simulink model "YMBOX_Control_Core"  (R2024b)
settings: Solver=FixedStepDiscrete  StartTime=0.0  StopTime=3  RelTol=1e-3
PreLoadFcn:
  | run(fullfile(fileparts(get_param(bdroot,'FileName')), 'YMBOX_Deluxe_init.m'));
InitFcn:
  | YMBOX_InitializeModel('core',bdroot);
model workspace (MAT data in the model file):
  KuMDAS_ObserverBuildVariant : Simulink.Parameter (value not decoded)
undefined symbols (not defined in the file or in its folder): CeMDSM_DrvModeIfStart_enum, CeMDSM_DrvModeSpdSens_enum, CeMDSM_DrvModeSpdSmo_enum, CeMDSM_DrvModeTrq_enum, Cf_CONTROL_TASK_TIME_S, KbMDAS_SmoDeadTimeCompEnable_flg, KbMDSA_ActiveInverterCompEnable_flg, KbMDSA_UnifiedVoltageLimitEnable_flg, KbMDSP_DCBusVoltReportFilterEnable_flg, KbMDTM_DAxisPriorityInFW_flg, KbMDTM_FieldWeakeningEnable_flg, KbMDTM_FinalIqAntiWindupEnable_flg, KbMDTM_SensorlessFieldWeakeningEnable_flg, KbMDTM_TorquePriorityBelowBase_flg, KbMDTM_UnifiedConstraintEnable_flg, KfMDAS_ControlCountToElecRad_NULL, KfMDAS_IfAccel_rpms, KfMDAS_IfAlignTime_s, KfMDAS_IfBlendTime_s, KfMDAS_IfSwitchSpd_rpm, KfMDAS_NativeCountToMechRad_NULL, KfMDAS_ObserverExitRatio_NULL, KfMDAS_SlsCtrlPeriod_s, KfMDAS_SlsEAngleInit_rad, KfMDAS_SlsElecSpdMax_rads, KfMDAS_SlsElecSpdMin_rads, KfMDAS_SlsTwoPi_rad, KfMDAS_SmoAngleOffset_rad, KfMDAS_SmoCurrentZohCoefA_NULL, KfMDAS_SmoCurrentZohCoefB_AperV, KfMDAS_SmoDeadTimeCurrentBoundary_A, KfMDAS_SmoDeadTimeDuty_NULL, KfMDAS_SmoDeadTimePolarity_NULL, KfMDAS_SmoDeviceDrop_V, KfMDAS_SmoEmfLpfCoefA_NULL, KfMDAS_SmoEmfLpfCoefB_NULL, KfMDAS_SmoEmfLpfInvPole_s, KfMDAS_SmoErrBoundaryMax_A, KfMDAS_SmoErrBoundarySpan_A, KfMDAS_SmoGainSchedAlpha_NULL, KfMDAS_SmoGainSchedAngleComp_rad, KfMDAS_SmoGainSchedEmfLow_V, KfMDAS_SmoGainSchedInvSpan_PerV, KfMDAS_SmoLdMinusLq_H, KfMDAS_SmoPllKiTs_NULL, KfMDAS_SmoPllKp_NULL, KfMDAS_SmoPllMinEmf_V, KfMDAS_SmoPllSpeedLpfAlpha_NULL, KfMDAS_SmoSlideGainMin_V, KfMDAS_SmoSlideGainSpan_V, KfMDAS_SmoSwitchSpd_rpm, KfMDAS_SmoTotalDelay_s, KfMDCC_DqSoftwareOverCurrentThreshold_A, KfMDCC_PiKcTsId_NULL, KfMDCC_PiKcTsIq_NULL, KfMDCC_PiKiTsId_NULL, KfMDCC_PiKiTsIq_NULL, KfMDCC_PiKpValueId_NULL, KfMDCC_PiKpValueIq_NULL, KfMDCC_PwmFreq_Hz ... (+84)
libraries: YMBOX_SharedMath_Lib x11, spsabctoAlphaBetaZeroLib x1
(part 6 of 8)

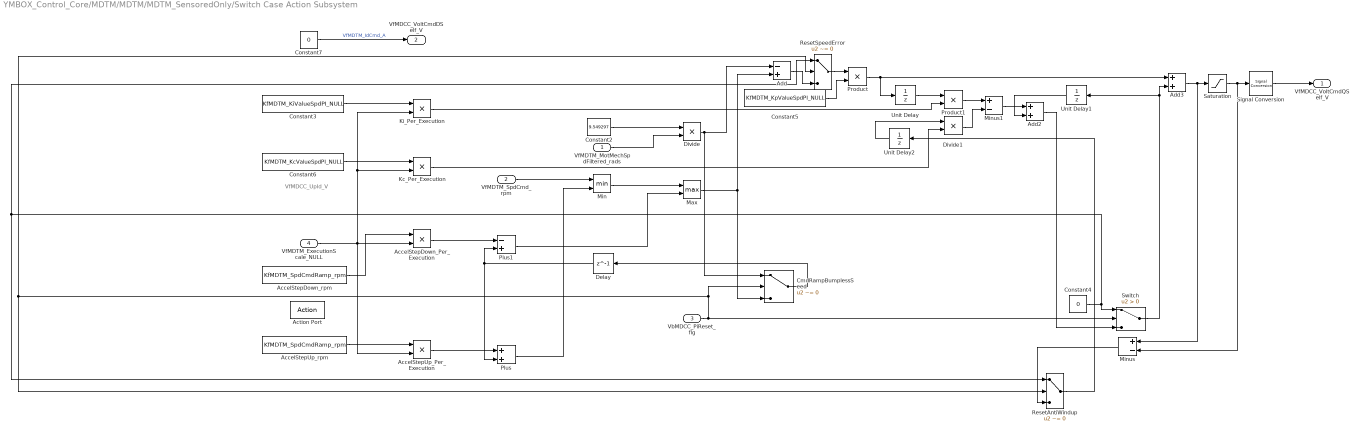
== system YMBOX_Control_Core/MDTM/MDTM/MDTM_SensoredOnly/Switch Case Action Subsystem ==
  note: VfMDCC_UpId_V
  VfMDTM_MotMechSpdFiltered_rads : Inport
  VfMDTM_SpdCmd_rpm : Inport  Port=2
  VbMDCC_PiReset_flg : Inport  Port=3
  VfMDTM_ExecutionScale_NULL : Inport  Port=4  OutDataTypeStr=single
  Action Port : ActionPort  InitializeStates=reset  ActionPortLabel=case [ 4 ]:
  AccelStepDown_Per_Execution : Product  Inputs=**
  AccelStepDown_rpm : Constant  Value=KfMDTM_SpdCmdRamp_rpm
  AccelStepUp_Per_Execution : Product  Inputs=**
  AccelStepUp_rpm : Constant  Value=KfMDTM_SpdCmdRamp_rpm
  Add : Sum  Inputs=-+
  Add2 : Sum  OutDataTypeStr=single
  Add3 : Sum
  CmdRampBumplessSeed : Switch  Criteria=u2 ~= 0  Threshold=0.5  SaturateOnIntegerOverflow=off  InputSameDT=off
  Constant2 : Constant  Value=9.549297  OutDataTypeStr=single
  Constant3 : Constant  Value=KfMDTM_KiValueSpdPI_NULL
  Constant4 : Constant  Value=0  OutDataTypeStr=single
  Constant5 : Constant  Value=KfMDTM_KpValueSpdPI_NULL
  Constant6 : Constant  Value=KfMDTM_KcValueSpdPI_NULL
  Constant7 : Constant  Value=0  OutDataTypeStr=single
  Delay : Delay  DelayLength=1
  Divide : Product  Inputs=**
  Divide1 : Product  Inputs=**
  Kc_Per_Execution : Product  Inputs=**
  Ki_Per_Execution : Product  Inputs=**
  Max : MinMax  Function=max  Inputs=2  OutDataTypeStr=single
  Min : MinMax  Inputs=2  OutDataTypeStr=single
  Minus : Sum  Inputs=+-
  Minus1 : Sum  Inputs=+-
  Plus : Sum
  Plus1 : Sum  Inputs=-+
  Product : Product
  Product1 : Product  RndMeth=Zero
  ResetAntiWindup : Switch  Criteria=u2 ~= 0
  ResetSpeedError : Switch  Criteria=u2 ~= 0
  Saturation : Saturate  UpperLimit=KfMDTM_IqCmdMax_A  LowerLimit=KfMDTM_IqCmdMin_A  OutDataTypeStr=single
  Signal Conversion : SignalConversion  OverrideOpt=off
  Switch : Switch  Criteria=u2 > Threshold  SaturateOnIntegerOverflow=off  InputSameDT=off
  Unit Delay : UnitDelay  SampleTime=-1  HasFrameUpgradeWarning=on
  Unit Delay1 : UnitDelay  SampleTime=-1  HasFrameUpgradeWarning=on
  Unit Delay2 : UnitDelay  SampleTime=-1  HasFrameUpgradeWarning=on
  VfMDCC_VoltCmdQSelf_V : Outport
  VfMDCC_VoltCmdDSelf_V : Outport  Port=2
  wires:
  Constant3/1 -> Ki_Per_Execution/1
  Kc_Per_Execution/1 -> Divide1/2
  Constant6/1 -> Kc_Per_Execution/1
  Constant7/1 -> VfMDCC_VoltCmdDSelf_V/1  "VfMDTM_IdCmd_A"
  VfMDTM_ExecutionScale_NULL/1 -> Ki_Per_Execution/2, Kc_Per_Execution/2, AccelStepDown_Per_Execution/2, AccelStepUp_Per_Execution/2
  AccelStepDown_rpm/1 -> AccelStepDown_Per_Execution/1
  Ki_Per_Execution/1 -> Product1/2
  AccelStepUp_rpm/1 -> AccelStepUp_Per_Execution/1
  AccelStepDown_Per_Execution/1 -> Plus1/1
  AccelStepUp_Per_Execution/1 -> Plus/1
  VfMDTM_SpdCmd_rpm/1 -> Min/1
  Plus1/1 -> Max/2
  Plus/1 -> Min/2
  Delay/1 -> Plus/2, Plus1/2
  Constant2/1 -> Divide/1
  VfMDTM_MotMechSpdFiltered_rads/1 -> Divide/2
  Min/1 -> Max/1
  Divide/1 -> CmdRampBumplessSeed/1, Add/1
  Max/1 -> CmdRampBumplessSeed/3, Add/2
  VbMDCC_PiReset_flg/1 -> ResetAntiWindup/2, ResetSpeedError/2, CmdRampBumplessSeed/2, Switch/2
  Add/1 -> ResetSpeedError/3
  Constant5/1 -> Product/2
  CmdRampBumplessSeed/1 -> Delay/1
  Product/1 -> Add3/1, Unit Delay/1
  Unit Delay2/1 -> Divide1/1
  Unit Delay/1 -> Product1/1
  Product1/1 -> Minus1/1
  Divide1/1 -> Minus1/2
  Minus1/1 -> Add2/1
  Add2/1 -> Switch/3
  Unit Delay1/1 -> Add2/2
  Constant4/1 -> ResetAntiWindup/1, ResetSpeedError/1, Switch/1
  Minus/1 -> ResetAntiWindup/3
  Switch/1 -> Add3/2, Unit Delay1/1
  Add3/1 -> Minus/1, Saturation/1
  Saturation/1 -> Signal Conversion/1, Minus/2
  Signal Conversion/1 -> VfMDCC_VoltCmdQSelf_V/1
  ResetSpeedError/1 -> Product/1
  ResetAntiWindup/1 -> Unit Delay2/1

== system YMBOX_Control_Core/MDTM/MDTM/MDTM_SensoredOnly/Switch Case Action Subsystem1 ==
  VfMDCC_TestUalphaUdId_NULL : Inport
  VfMDTM_TestUbetaUqIq_NULL : Inport  Port=2
  Action Port : ActionPort  ActionPortLabel=case [ 3 ]:
  Iq : Outport
  Id : Outport  Port=2
  wires:
  VfMDCC_TestUalphaUdId_NULL/1 -> Id/1
  VfMDTM_TestUbetaUqIq_NULL/1 -> Iq/1

== system YMBOX_Control_Core/MDTM/MDTM/MDTM_SensoredOnly/Switch Case Action Subsystem2 ==
  VfMDTM_TrqCmd_Nm : Inport
  Action Port : ActionPort  ActionPortLabel=case [ 5 ]:
  Constant7 : Constant  Value=0  OutDataTypeStr=single
  Gain : Gain  Gain=KfMDTM_Trq2Iq_NULL
  Iq : Outport
  Id : Outport  Port=2
  wires:
  Gain/1 -> Iq/1
  Constant7/1 -> Id/1  "VfMDTM_IdCmd_A"
  VfMDTM_TrqCmd_Nm/1 -> Gain/1

== system YMBOX_Control_Core/MDAS/MDAS_DriveModeRoute_Variant/MDAS_Route_SMO/Switch Case Action Subsystem/Switch Case Action Subsystem6 ==
  In1 : Inport
  Action Port : ActionPort  ActionPortLabel=if(u1 > KfPLL_HalfPositionCounts_NULL)
  Constant : Constant  Value=KfPLL_PositionCountsPerRev_NULL
  Minus : Sum  Inputs=+-
  Out1 : Outport
  wires:
  In1/1 -> Minus/1
  Constant/1 -> Minus/2
  Minus/1 -> Out1/1

== system YMBOX_Control_Core/MDAS/MDAS_DriveModeRoute_Variant/MDAS_Route_SMO/Switch Case Action Subsystem/Switch Case Action Subsystem7 ==
  In1 : Inport
  Action Port : ActionPort  ActionPortLabel=elseif(u1 < -KfPLL_HalfPositionCounts_NULL)
  Constant : Constant  Value=KfPLL_PositionCountsPerRev_NULL
  Minus : Sum
  Out1 : Outport
  wires:
  Minus/1 -> Out1/1
  In1/1 -> Minus/1
  Constant/1 -> Minus/2

== system YMBOX_Control_Core/MDAS/MDAS_DriveModeRoute_Variant/MDAS_Route_SMO/Switch Case Action Subsystem/Switch Case Action Subsystem8 ==
  In1 : Inport
  Action Port : ActionPort  ActionPortLabel=else
  Out1 : Outport
  wires:
  In1/1 -> Out1/1

== system YMBOX_Control_Core/MDAS/MDAS_DriveModeRoute_Variant/MDAS_Route_SensoredOnly/Sensored_AngleSpeed/Switch Case Action Subsystem6 ==
  In1 : Inport
  Action Port : ActionPort  ActionPortLabel=if(u1 > KfPLL_HalfPositionCounts_NULL)
  Constant : Constant  Value=KfPLL_PositionCountsPerRev_NULL
  Minus : Sum  Inputs=+-
  Out1 : Outport
  wires:
  Minus/1 -> Out1/1
  Constant/1 -> Minus/2
  In1/1 -> Minus/1

== system YMBOX_Control_Core/MDAS/MDAS_DriveModeRoute_Variant/MDAS_Route_SensoredOnly/Sensored_AngleSpeed/Switch Case Action Subsystem7 ==
  In1 : Inport
  Action Port : ActionPort  ActionPortLabel=elseif(u1 < -KfPLL_HalfPositionCounts_NULL)
  Constant : Constant  Value=KfPLL_PositionCountsPerRev_NULL
  Minus : Sum
  Out1 : Outport
  wires:
  Constant/1 -> Minus/2
  In1/1 -> Minus/1
  Minus/1 -> Out1/1

== system YMBOX_Control_Core/MDAS/MDAS_DriveModeRoute_Variant/MDAS_Route_SensoredOnly/Sensored_AngleSpeed/Switch Case Action Subsystem8 ==
  In1 : Inport
  Action Port : ActionPort  ActionPortLabel=else
  Out1 : Outport
  wires:
  In1/1 -> Out1/1

== system YMBOX_Control_Core/MDAS/Sensorless_FluxMRAS/Observer_Variant1_SMO/SMO_Observer/ExtendedEmfVoltageModel ==
  currentAb0_A : Inport
  appliedVoltageAb0_V : Inport  Port=2
  estimatedSpeed_rads : Inport  Port=3
  AlphaCrossCoupling : Product  Inputs=**
  BetaCrossCoupling : Product  Inputs=**
  CurrentAlphaBetaZero : Demux  Outputs=3
  EquivalentVoltageAb0 : Mux  Inputs=3
  ExtendedVoltageAlpha : Sum  Inputs=+-
  ExtendedVoltageBeta : Sum  Inputs=|++
  PreviousEstimatedSpeed : UnitDelay  InitialCondition=single(0)  SampleTime=-1
  PreviousMeasuredCurrent : UnitDelay  InitialCondition=single(0)  SampleTime=-1
  SpeedTimesLdMinusLq : Gain  Gain=KfMDAS_SmoLdMinusLq_H
  UnusedZeroSequenceCurrent : Terminator
  VoltageAlphaBetaZero : Demux  Outputs=3
  equivalentVoltageAb0_V : Outport
  wires:
  estimatedSpeed_rads/1 -> PreviousEstimatedSpeed/1
  appliedVoltageAb0_V/1 -> VoltageAlphaBetaZero/1
  CurrentAlphaBetaZero/2 -> AlphaCrossCoupling/2
  PreviousMeasuredCurrent/1 -> CurrentAlphaBetaZero/1
  currentAb0_A/1 -> PreviousMeasuredCurrent/1
  PreviousEstimatedSpeed/1 -> SpeedTimesLdMinusLq/1
  CurrentAlphaBetaZero/1 -> BetaCrossCoupling/2
  SpeedTimesLdMinusLq/1 -> BetaCrossCoupling/1, AlphaCrossCoupling/1
  CurrentAlphaBetaZero/3 -> UnusedZeroSequenceCurrent/1
  AlphaCrossCoupling/1 -> ExtendedVoltageAlpha/2
  BetaCrossCoupling/1 -> ExtendedVoltageBeta/2
  VoltageAlphaBetaZero/1 -> ExtendedVoltageAlpha/1
  VoltageAlphaBetaZero/2 -> ExtendedVoltageBeta/1
  VoltageAlphaBetaZero/3 -> EquivalentVoltageAb0/3
  ExtendedVoltageAlpha/1 -> EquivalentVoltageAb0/1
  ExtendedVoltageBeta/1 -> EquivalentVoltageAb0/2
  EquivalentVoltageAb0/1 -> equivalentVoltageAb0_V/1

== system YMBOX_Control_Core/MDAS/Sensorless_FluxMRAS/Observer_Variant1_SMO/SMO_Observer/PLL_Speed_Output ==
  IntegralSpeed_rads : Inport
  ProportionalCorrection_rads : Inport  Port=2
  CorrectedSpeed : Sum  OutDataTypeStr=single
  FilteredProportionalCorrection : Sum  OutDataTypeStr=single
  PreviousProportionalCorrection : UnitDelay  InitialCondition=single(0)  SampleTime=-1
  ProportionalFilterCoefficient : Gain  Gain=KfMDAS_SmoPllSpeedLpfAlpha_NULL  OutDataTypeStr=single
  ProportionalFilterError : Sum  Inputs=+-  OutDataTypeStr=single
  SpeedLimit : Saturate  UpperLimit=KfMDAS_SlsElecSpdMax_rads  LowerLimit=KfMDAS_SlsElecSpdMin_rads  OutDataTypeStr=single
  Speed_rads : Outport
  wires:
  CorrectedSpeed/1 -> SpeedLimit/1
  ProportionalCorrection_rads/1 -> ProportionalFilterError/1
  ProportionalFilterCoefficient/1 -> FilteredProportionalCorrection/1
  ProportionalFilterError/1 -> ProportionalFilterCoefficient/1
  PreviousProportionalCorrection/1 -> FilteredProportionalCorrection/2, ProportionalFilterError/2
  IntegralSpeed_rads/1 -> CorrectedSpeed/1
  FilteredProportionalCorrection/1 -> PreviousProportionalCorrection/1, CorrectedSpeed/2
  SpeedLimit/1 -> Speed_rads/1

== system YMBOX_Control_Core/MDAS/Sensorless_FluxMRAS/Observer_Variant1_SMO/SMO_Observer/SMO_SinCos_Adapter ==
  thetaRad : Inport
  twoPiRad : Inport  Port=2
  AnglePu_To_Single : DataTypeConversion  OutDataTypeStr=single
  Cos_To_ObserverType : DataTypeConversion  OutDataTypeStr=single
  SinCos_Service : YMBOX_SharedMath_Lib/SinCos_Service  SystemSampleTime=-1  VariantActivationTime=update diagram  AllowFlexibleInterface=on  Latency=0  AutoFrameSizeCalculation=off
  Sin_To_ObserverType : DataTypeConversion  OutDataTypeStr=single
  ThetaRad_To_Pu : Product  Inputs=*/
  cosTheta : Outport
  sinTheta : Outport  Port=2
  wires:
  Cos_To_ObserverType/1 -> cosTheta/1
  SinCos_Service/2 -> Sin_To_ObserverType/1
  thetaRad/1 -> ThetaRad_To_Pu/1
  twoPiRad/1 -> ThetaRad_To_Pu/2
  Sin_To_ObserverType/1 -> sinTheta/1
  SinCos_Service/1 -> Cos_To_ObserverType/1
  ThetaRad_To_Pu/1 -> AnglePu_To_Single/1
  AnglePu_To_Single/1 -> SinCos_Service/1

== system YMBOX_Control_Core/MDCC/MDCC_Subsystem/DqSoftwareOverCurrent_Diagnostic/CountWhenDqCurrentExceeded/AssertDqSoftwareOverCurrent ==
  Action Port : ActionPort  ActionPortLabel=else
  TRUE : Constant  OutDataTypeStr=boolean
  VbMDCC_DqSoftwareOverCurrent_flg : Outport  OutputWhenDisabled=reset  InitialOutput=false
  wires:
  TRUE/1 -> VbMDCC_DqSoftwareOverCurrent_flg/1

== system YMBOX_Control_Core/MDCC/MDCC_Subsystem/DqSoftwareOverCurrent_Diagnostic/CountWhenDqCurrentExceeded/IncrementDqSoftwareOverCurrentCount ==
  VuMDCC_DqSoftwareOverCurrentCount_cnt : Inport
  Action Port : ActionPort  ActionPortLabel=if(u1<u2)
  Constant : Constant  OutDataTypeStr=uint8
  Sum : Sum  OutDataTypeStr=uint8
  VuMDCC_DqSoftwareOverCurrentCountNew_cnt : Outport
  wires:
  VuMDCC_DqSoftwareOverCurrentCount_cnt/1 -> Sum/1
  Constant/1 -> Sum/2
  Sum/1 -> VuMDCC_DqSoftwareOverCurrentCountNew_cnt/1

== system YMBOX_Control_Core/MDCC/MDCC_Subsystem/DqSoftwareOverCurrent_Diagnostic/CountWhenDqCurrentNormal/DecrementDqSoftwareOverCurrentCount ==
  VuMDCC_DqSoftwareOverCurrentCount_cnt : Inport
  Action Port : ActionPort  ActionPortLabel=if(u1~=0)
  Constant : Constant  OutDataTypeStr=uint8
  Sum : Sum  Inputs=+-  OutDataTypeStr=uint8
  VuMDCC_DqSoftwareOverCurrentCountNew_cnt : Outport
  wires:
  Sum/1 -> VuMDCC_DqSoftwareOverCurrentCountNew_cnt/1
  Constant/1 -> Sum/2
  VuMDCC_DqSoftwareOverCurrentCount_cnt/1 -> Sum/1

== system YMBOX_Control_Core/MDCC/MDCC_Subsystem/UdUqCalc/UdUqCalc/PI_Id_Self ==
  note: VfMDCC_UpId_V
  VfMDCC_DCurCmd_A : Inport
  VfMDCC_DCur_A : Inport  Port=2
  VfMDCC_PiKpValueId_NULL : Inport  Port=3
  VbMDCC_PiReset_flg : Inport  Port=4
  VfMDCC_k_effective_NULL : Inport  Port=5
  Add : Sum  Inputs=+-
  Add1 : Sum
  Add2 : Sum  OutDataTypeStr=single
  Add3 : Sum
  Constant : Constant  Value=KfMDCC_PiKiTsId_NULL
  Constant1 : Constant  Value=KfMDCC_PiKcTsId_NULL
  Constant2 : Constant  Value=0  OutDataTypeStr=single
  Constant3 : Constant  OutDataTypeStr=single
  Delay : Delay  DelayLength=1  InputProcessing=Columns as channels (frame based)
  Divide2 : Product  Inputs=**
  Plus : Sum  Inputs=-+
  Product : Product
  Product1 : Product  RndMeth=Zero
  Product2 : Product  OutDataTypeStr=single  RndMeth=Zero
  Switch : Switch  Criteria=u2 > Threshold  SaturateOnIntegerOverflow=off  InputSameDT=off
  Unit Delay : UnitDelay  SampleTime=-1  HasFrameUpgradeWarning=on
  Unit Delay1 : UnitDelay  SampleTime=-1  HasFrameUpgradeWarning=on
  VfMDCC_VoltCmdDSelf_V : Outport
  wires:
  Divide2/1 -> Product2/1
  Plus/1 -> Divide2/2
  Constant3/1 -> Plus/1
  VfMDCC_k_effective_NULL/1 -> Plus/2
  Delay/1 -> Divide2/1
  Add2/1 -> Switch/3
  VbMDCC_PiReset_flg/1 -> [VbMDCC_PiReset_flg]
  Switch/1 -> Unit Delay1/1, Add3/2
  Constant2/1 -> Switch/1
  [VbMDCC_PiReset_flg] -> Switch/2
  Constant1/1 -> Product2/2
  Add3/1 -> VfMDCC_VoltCmdDSelf_V/1, Delay/1
  Unit Delay1/1 -> Add2/2
  Add1/1 -> Add2/1
  Constant/1 -> Product1/2
  Unit Delay/1 -> Product1/1
  Product/1 -> Add3/1, Unit Delay/1
  VfMDCC_PiKpValueId_NULL/1 -> Product/2
  Add/1 -> Product/1
  VfMDCC_DCur_A/1 -> Add/2
  VfMDCC_DCurCmd_A/1 -> Add/1
  Product1/1 -> Add1/1
  Product2/1 -> Add1/2

== system YMBOX_Control_Core/MDCC/MDCC_Subsystem/UdUqCalc/UdUqCalc/PI_Iq_Self ==
  note: VfMDCC_UpIq_V
  VfMDCC_QCurCmd_A : Inport
  VfMDCC_QCur_A : Inport  Port=2
  VfMDCC_PiKpValueIq_NULL : Inport  Port=3
  VbMDCC_PiReset_flg : Inport  Port=4
  VfMDCC_k_effective_NULL : Inport  Port=5
  Add : Sum  Inputs=+-
  Add1 : Sum  OutDataTypeStr=single
  Add2 : Sum  OutDataTypeStr=single
  Add3 : Sum
  Constant : Constant  Value=KfMDCC_PiKiTsIq_NULL
  Constant1 : Constant  Value=KfMDCC_PiKcTsIq_NULL
  Constant2 : Constant  Value=0  OutDataTypeStr=single
  Constant3 : Constant  OutDataTypeStr=single
  Delay : Delay  DelayLength=1  InputProcessing=Columns as channels (frame based)
  Divide2 : Product  Inputs=**
  Plus : Sum  Inputs=-+
  Product : Product
  Product1 : Product  RndMeth=Zero
  Product2 : Product  OutDataTypeStr=single  RndMeth=Zero
  Switch : Switch  Criteria=u2 > Threshold  SaturateOnIntegerOverflow=off  InputSameDT=off
  Unit Delay : UnitDelay  SampleTime=-1  HasFrameUpgradeWarning=on
  Unit Delay1 : UnitDelay  SampleTime=-1  HasFrameUpgradeWarning=on
  VfMDCC_VoltCmdQSelf_V : Outport
  wires:
  Plus/1 -> Divide2/2
  Divide2/1 -> Product2/1
  VfMDCC_k_effective_NULL/1 -> Plus/2
  Constant3/1 -> Plus/1
  Delay/1 -> Divide2/1
  Switch/1 -> Unit Delay1/1, Add3/2
  Add2/1 -> Switch/3
  Constant2/1 -> Switch/1
  [VbMDCC_PiReset_flg] -> Switch/2
  VbMDCC_PiReset_flg/1 -> [VbMDCC_PiReset_flg]
  Constant1/1 -> Product2/2
  Add3/1 -> Delay/1, VfMDCC_VoltCmdQSelf_V/1
  Unit Delay1/1 -> Add2/2
  Add1/1 -> Add2/1
  Constant/1 -> Product1/2
  Unit Delay/1 -> Product1/1
  Product/1 -> Add3/1, Unit Delay/1
  VfMDCC_PiKpValueIq_NULL/1 -> Product/2
  Add/1 -> Product/1
  VfMDCC_QCur_A/1 -> Add/2
  VfMDCC_QCurCmd_A/1 -> Add/1
  Product1/1 -> Add1/1
  Product2/1 -> Add1/2

== system YMBOX_Control_Core/MDCC/MDCC_Subsystem/UdUqCalc/UdUqCalc/Switch Case Action Subsystem ==
  VfMDCC_VoltCmdDSelf_V : Inport
  VfMDCC_VoltCmdQSelf_V : Inport  Port=2
  Action Port : ActionPort  ActionPortLabel=case [ 0 ]:
  VfMDCC_VoltD_V : Outport
  VfMDCC_VoltQ_V : Outport  Port=2
  wires:
  VfMDCC_VoltCmdDSelf_V/1 -> VfMDCC_VoltD_V/1
  VfMDCC_VoltCmdQSelf_V/1 -> VfMDCC_VoltQ_V/1

== system YMBOX_Control_Core/MDCC/MDCC_Subsystem/UdUqCalc/UdUqCalc/Switch Case Action Subsystem1 ==
  VfMDCC_VoltCmdDSelf_V : Inport
  VfMDCC_VoltCmdQSelf_V : Inport  Port=2
  VfMDCC_DCur_A : Inport  Port=3
  VfMDCC_QCur_A : Inport  Port=4
  VfMDCC_MotESpdFiltered_rads : Inport  Port=5
  Action Port : ActionPort  ActionPortLabel=case [ 1 ]:
  Add : Sum
  Add1 : Sum
  Add2 : Sum  Inputs=+-
  Constant : Constant  Value=KfMDMP_EquiInductanceValueD_H
  Constant1 : Constant  Value=KfMDMP_EquiFluxValue_Wb
  Constant2 : Constant  Value=KfMDCC_VqFFScale_NULL
  Constant3 : Constant  Value=KfMDMP_EquiInductanceValueQ_H
  Constant4 : Constant  Value=KfMDCC_VdFFScale_NULL
  Product{,1..2,5} (4 alike) : Product
  Product3 : Product  RndMeth=Zero
  Product4 : Product  RndMeth=Zero
  VfMDCC_VoltD_V : Outport
  VfMDCC_VoltQ_V : Outport  Port=2
  wires:
  Constant/1 -> Product/1
  Constant1/1 -> Add/2
  Constant3/1 -> Product3/2
  Product4/1 -> Product5/1
  Add1/1 -> VfMDCC_VoltQ_V/1
  Product1/1 -> Product2/1
  Constant4/1 -> Product5/2
  Constant2/1 -> Product2/2
  VfMDCC_VoltCmdQSelf_V/1 -> Add1/1
  Product5/1 -> Add2/2
  VfMDCC_DCur_A/1 -> Product/2
  Product/1 -> Add/1
  VfMDCC_QCur_A/1 -> Product3/1
  Add/1 -> Product1/2
  Add2/1 -> VfMDCC_VoltD_V/1
  VfMDCC_MotESpdFiltered_rads/1 -> Product4/2, Product1/1
  Product3/1 -> Product4/1
  Product2/1 -> Add1/2
  VfMDCC_VoltCmdDSelf_V/1 -> Add2/1

== system YMBOX_Control_Core/MDCC/MDCC_Subsystem/UdUqCalc/UdUqCalc/Switch Case Action Subsystem2 ==
  VfMDCC_VoltCmdDSelf_V : Inport
  VfMDCC_VoltCmdQSelf_V : Inport  Port=2
  VfMDCC_QCur_A : Inport  Port=3
  VfMDCC_MotESpdFiltered_rads : Inport  Port=4
  Action Port : ActionPort  ActionPortLabel=case [ 2 ]:
  Add2 : Sum  Inputs=+-
  Constant3 : Constant  Value=KfMDMP_EquiInductanceValueQ_H
  Constant4 : Constant  Value=KfMDCC_VdFFScale_NULL
  Product3 : Product  RndMeth=Zero
  Product4 : Product  RndMeth=Zero
  Product5 : Product
  VfMDCC_VoltD_V : Outport
  VfMDCC_VoltQ_V : Outport  Port=2
  wires:
  Product4/1 -> Product5/1
  VfMDCC_VoltCmdDSelf_V/1 -> Add2/1
  VfMDCC_VoltCmdQSelf_V/1 -> VfMDCC_VoltQ_V/1
  Constant3/1 -> Product3/2
  Product5/1 -> Add2/2
  Product3/1 -> Product4/1
  VfMDCC_MotESpdFiltered_rads/1 -> Product4/2
  Add2/1 -> VfMDCC_VoltD_V/1
  VfMDCC_QCur_A/1 -> Product3/1
  Constant4/1 -> Product5/2

== system YMBOX_Control_Core/MDCC/MDCC_Subsystem/UdUqCalc/UdUqCalc/Switch Case Action Subsystem3 ==
  VfMDCC_VoltCmdDSelf_V : Inport
  VfMDCC_VoltCmdQSelf_V : Inport  Port=2
  VfMDCC_DCur_A : Inport  Port=3
  VfMDCC_MotESpdFiltered_rads : Inport  Port=4
  Action Port : ActionPort  ActionPortLabel=case [ 3 ]:
  Add : Sum
  Add1 : Sum
  Constant : Constant  Value=KfMDMP_EquiInductanceValueD_H
  Constant1 : Constant  Value=KfMDMP_EquiFluxValue_Wb
  Constant2 : Constant  Value=KfMDCC_VqFFScale_NULL
  Product : Product
  Product1 : Product
  Product2 : Product
  VfMDCC_VoltD_V : Outport
  VfMDCC_VoltQ_V : Outport  Port=2
  wires:
  VfMDCC_MotESpdFiltered_rads/1 -> Product1/1
  VfMDCC_DCur_A/1 -> Product/2
  Product/1 -> Add/1
  Add1/1 -> VfMDCC_VoltQ_V/1
  Product1/1 -> Product2/1
  VfMDCC_VoltCmdQSelf_V/1 -> Add1/1
  Constant1/1 -> Add/2
  Constant/1 -> Product/1
  Product2/1 -> Add1/2
  VfMDCC_VoltCmdDSelf_V/1 -> VfMDCC_VoltD_V/1
  Add/1 -> Product1/2
  Constant2/1 -> Product2/2

== system YMBOX_Control_Core/MDSA/MDSA_Subsystem/PwmOutput/PwmEnable/SVM ==
  VfMDSA_VoltAlpha_V : Inport
  VfMDSA_VoltBeta_V : Inport  Port=2
  VfMDSA_DCBusVolt_V : Inport  Port=3
  SectorCalc : Subsystem  RTWFcnName=vPwm_MDSA_SVM_SectorCalc  RTWFileName=MDSA
      settings: RTWSystemCode=Nonreusable function  RTWFcnNameOpts=User specified  RTWFileNameOpts=User specified
  T1T2CoefCalc : Subsystem  RTWFcnName=vPwm_MDSA_SVM_T1T2CoefCalc  RTWFileName=MDSA
      settings: RTWSystemCode=Nonreusable function  RTWFcnNameOpts=User specified  RTWFileNameOpts=User specified
  TonUVWCal : Subsystem  RTWFcnName=vPwm_MDSA_SVM_TonUVWCalc  RTWFileName=MDSA
      settings: RTWSystemCode=Nonreusable function  RTWFcnNameOpts=User specified  RTWFileNameOpts=User specified
  VfMDSA_PwmDutyCyclePhaseU_NULL : Outport
  VfMDSA_PwmDutyCyclePhaseV_NULL : Outport  Port=2
  VfMDSA_PwmDutyCyclePhaseW_NULL : Outport  Port=3
  VfMDSA_k_svm_NULL : Outport  Port=4
  wires:
  T1T2CoefCalc/3(VfMDSA_k_svm_NULL) -> VfMDSA_k_svm_NULL/1
  TonUVWCal/1(VfMDSA_PwmDutyCyclePhaseU_NULL) -> VfMDSA_PwmDutyCyclePhaseU_NULL/1
  TonUVWCal/3(VfMDSA_PwmDutyCyclePhaseW_NULL) -> VfMDSA_PwmDutyCyclePhaseW_NULL/1
  TonUVWCal/2(VfMDSA_PwmDutyCyclePhaseV_NULL) -> VfMDSA_PwmDutyCyclePhaseV_NULL/1
  SectorCalc/1(VeMDSA_Sector_enum) -> TonUVWCal/1(VeMDSA_Sector_enum), T1T2CoefCalc/1(VeMDSA_Sector_enum)
  T1T2CoefCalc/2(VfMDSA_T2Coef_NULL) -> TonUVWCal/3(VfMDSA_T2Coef_NULL)
  T1T2CoefCalc/1(VfMDSA_T1Coef_NULL) -> TonUVWCal/2(VfMDSA_T1Coef_NULL)
  VfMDSA_DCBusVolt_V/1 -> T1T2CoefCalc/4(VfMDSA_DCBusVolt_V)
  VfMDSA_VoltBeta_V/1 -> SectorCalc/2(VfMDSA_VoltBeta_V), T1T2CoefCalc/3(VfMDSA_VoltBeta_V)
  VfMDSA_VoltAlpha_V/1 -> SectorCalc/1(VfMDSA_VoltAlpha_V), T1T2CoefCalc/2(VfMDSA_VoltAlpha_V)

== system YMBOX_Control_Core/MDSA/MDSA_Subsystem/UalphaUbetaCalc/Subsystem/UalphaUbetaCalc1 ==
  VfMDSA_VoltD_V : Inport
  VfMDSA_VoltQ_V : Inport  Port=2
  VfMDSA_MotElecAngle_rad : Inport  Port=3
  VfMDSA_MotElecSpd_rads : Inport  Port=4
  VfMDSA_PwmFreq_Hz : Inport  Port=5
  Action Port : ActionPort  ActionPortLabel=default:
  ElecAngle_Advance_SinCos : Subsystem  TreatAsAtomicUnit=on  RTWFcnName=vPwm_MDSA_UalphaUbetaCalc1_LookUpEAngleEstimatedCosSin  RTWFileName=MDSA
      settings: RTWFcnNameOpts=User specified  RTWFileNameOpts=User specified
  IPark : Subsystem  TreatAsAtomicUnit=on  RTWFcnName=vPwm_MDSA_UalphaUbetaCalc1_IPark  RTWFileName=MDSA
      settings: RTWFcnNameOpts=User specified  RTWFileNameOpts=User specified
  VfMDSA_VoltAlpha_V : Outport
  VfMDSA_VoltBeta_V : Outport  Port=2
  wires:
  VfMDSA_PwmFreq_Hz/1 -> ElecAngle_Advance_SinCos/3(VfMDSA_PwmFreq_Hz)
  IPark/2(VfMDSA_VoltBeta_V) -> VfMDSA_VoltBeta_V/1
  IPark/1(VfMDSA_VoltAlpha_V) -> VfMDSA_VoltAlpha_V/1
  VfMDSA_VoltD_V/1 -> IPark/1(VfMDSA_VoltD_V)  "VfMDSA_VoltD_V"
  VfMDSA_VoltQ_V/1 -> IPark/2(VfMDSA_VoltQ_V)  "VfMDSA_VoltQ_V"
  ElecAngle_Advance_SinCos/2(VfMDSA_EAngleEstimatedSin_NULL) -> IPark/4(VfMDSA_EAngleEstimatedSin_NULL)
  ElecAngle_Advance_SinCos/1(VfMDSA_EAngleEstimatedCos_NULL) -> IPark/3(VfMDSA_EAngleEstimatedCos_NULL)
  VfMDSA_MotElecSpd_rads/1 -> ElecAngle_Advance_SinCos/2(VfMDSA_MotElecSpd_rads)
  VfMDSA_MotElecAngle_rad/1 -> ElecAngle_Advance_SinCos/1(VfMDSA_MotElecAngle_rad)

== system YMBOX_Control_Core/MDSA/MDSA_Subsystem/UalphaUbetaCalc/Subsystem/UalphaUbetaCalc2 ==
  VfMDSA_TestUalphaUdId_NULL : Inport
  VfMDSA_TestUbetaUqIq_NULL : Inport  Port=2
  Action Port : ActionPort  ActionPortLabel=case [ 1 ]:
  VfMDSA_VoltAlpha_V : Outport
  VfMDSA_VoltBeta_V : Outport  Port=2
  wires:
  VfMDSA_TestUbetaUqIq_NULL/1 -> VfMDSA_VoltBeta_V/1
  VfMDSA_TestUalphaUdId_NULL/1 -> VfMDSA_VoltAlpha_V/1

== system YMBOX_Control_Core/MDTM/MDTM/MDTM_SMO/SMO_Handover_Current_Comp/Current_Vector_Crossfade ==
  sourceId : Inport  OutDataTypeStr=single
  sourceIq : Inport  Port=2  OutDataTypeStr=single
  currentWeight : Inport  Port=3  OutDataTypeStr=single
  targetId : Inport  Port=4  OutDataTypeStr=single
  targetIq : Inport  Port=5  OutDataTypeStr=single
  Active_Blend_Enable : EnablePort  OutDataTypeStr=boolean
  Blend_Id : Sum  Inputs=|++
  Blend_Iq : Sum  Inputs=|++
  One_Minus_Current_Weight : Sum  Inputs=+-
  Unity : Constant  Value=single(1)
  Weighted_Source_Id : Product  Inputs=**
  Weighted_Source_Iq : Product  Inputs=**
  Weighted_Target_Id : Product  Inputs=**
  Weighted_Target_Iq : Product  Inputs=**
  idBlend : Outport  OutDataTypeStr=single
  iqBlend : Outport  Port=2  OutDataTypeStr=single
  wires:
  Blend_Iq/1 -> iqBlend/1
  Blend_Id/1 -> idBlend/1
  Weighted_Target_Iq/1 -> Blend_Iq/2
  Weighted_Source_Iq/1 -> Blend_Iq/1
  targetIq/1 -> Weighted_Target_Iq/1
  sourceIq/1 -> Weighted_Source_Iq/1
  Weighted_Target_Id/1 -> Blend_Id/2
  Weighted_Source_Id/1 -> Blend_Id/1
  targetId/1 -> Weighted_Target_Id/1
  One_Minus_Current_Weight/1 -> Weighted_Source_Id/2, Weighted_Source_Iq/2
  sourceId/1 -> Weighted_Source_Id/1
  currentWeight/1 -> One_Minus_Current_Weight/2, Weighted_Target_Id/2, Weighted_Target_Iq/2
  Unity/1 -> One_Minus_Current_Weight/1

== system YMBOX_Control_Core/MDTM/MDTM/MDTM_SMO/SMO_Handover_Current_Comp/Handover_Enable_Logic ==
  modeCmd : Inport  OutDataTypeStr=uint16
  modeReq : Inport  Port=2  OutDataTypeStr=uint16
  blendWeight : Inport  Port=3  OutDataTypeStr=single
  Blend_Complete : Constant  Value=single(1)
  Enable_Active_Blend : Logic  Inputs=3  IconShape=distinctive
  Is_Blend_Incomplete : RelationalOperator  Operator=<
  Is_Mode_17 : RelationalOperator  Operator===
  Is_Request_6 : RelationalOperator  Operator===
  Mode_SMO_ClosedLoop : Constant  Value=uint16(17)
  Request_Product_SMO : Constant  Value=uint16(6)
  activeBlend : Outport  OutDataTypeStr=boolean
  wires:
  Enable_Active_Blend/1 -> activeBlend/1
  Is_Blend_Incomplete/1 -> Enable_Active_Blend/3
  Is_Request_6/1 -> Enable_Active_Blend/2
  Is_Mode_17/1 -> Enable_Active_Blend/1
  Blend_Complete/1 -> Is_Blend_Incomplete/2
  blendWeight/1 -> Is_Blend_Incomplete/1
  Request_Product_SMO/1 -> Is_Request_6/2
  modeReq/1 -> Is_Request_6/1
  Mode_SMO_ClosedLoop/1 -> Is_Mode_17/2
  modeCmd/1 -> Is_Mode_17/1

== system YMBOX_Control_Core/MDTM/MDTM/MDTM_SMO/SMO_Handover_Current_Comp/Source_Frame_Rotation ==
  sourceId0 : Inport  OutDataTypeStr=single
  sourceIq0 : Inport  Port=2  OutDataTypeStr=single
  blendWeight : Inport  Port=3  OutDataTypeStr=single
  elecAngleDeltaRad : Inport  Port=4  OutDataTypeStr=single
  Active_Blend_Enable : EnablePort  OutDataTypeStr=boolean
  Id_Cos : Product  Inputs=**
  Id_Sin : Product  Inputs=**
  Iq_Cos : Product  Inputs=**
  Iq_Sin : Product  Inputs=**
  Rotated_Source_Id : Sum  Inputs=+-
  Rotated_Source_Iq : Sum  Inputs=|++
  SourcePhase_PU_Floor : Rounding
  SourcePhase_PU_Wrap : Sum  Inputs=+-
  SourcePhase_RadToPU : Gain  Gain=single(0.15915494)
  SourcePhase_SinCos_Service : YMBOX_SharedMath_Lib/SinCos_Service  SystemSampleTime=-1  VariantActivationTime=update diagram  AllowFlexibleInterface=on  Latency=0  AutoFrameSizeCalculation=off
  Source_Phase : Product  Inputs=**
  sourceId : Outport  OutDataTypeStr=single
  sourceIq : Outport  Port=2  OutDataTypeStr=single
  wires:
  blendWeight/1 -> Source_Phase/1
  SourcePhase_PU_Wrap/1 -> SourcePhase_SinCos_Service/1
  elecAngleDeltaRad/1 -> Source_Phase/2
  SourcePhase_RadToPU/1 -> SourcePhase_PU_Wrap/1, SourcePhase_PU_Floor/1
  Source_Phase/1 -> SourcePhase_RadToPU/1
  sourceIq0/1 -> Iq_Sin/1, Iq_Cos/1
  sourceId0/1 -> Id_Cos/1, Id_Sin/1
  SourcePhase_SinCos_Service/1 -> Iq_Cos/2, Id_Cos/2
  SourcePhase_SinCos_Service/2 -> Id_Sin/2, Iq_Sin/2
  Id_Sin/1 -> Rotated_Source_Iq/1
  Iq_Cos/1 -> Rotated_Source_Iq/2
  Id_Cos/1 -> Rotated_Source_Id/1
  Iq_Sin/1 -> Rotated_Source_Id/2
  Rotated_Source_Iq/1 -> sourceIq/1
  Rotated_Source_Id/1 -> sourceId/1
  SourcePhase_PU_Floor/1 -> SourcePhase_PU_Wrap/2

== system YMBOX_Control_Core/MDTM/MDTM/MDTM_SMO/SMO_Handover_Current_Comp/Target_Frame_Rotation ==
  idRaw : Inport  OutDataTypeStr=single
  iqRaw : Inport  Port=2  OutDataTypeStr=single
  blendWeight : Inport  Port=3  OutDataTypeStr=single
  elecAngleDeltaRad : Inport  Port=4  OutDataTypeStr=single
  Active_Blend_Enable : EnablePort  OutDataTypeStr=boolean
  Id_Cos : Product  Inputs=**
  Id_Sin : Product  Inputs=**
  Iq_Cos : Product  Inputs=**
  Iq_Sin : Product  Inputs=**
  One_Minus_Blend : Sum  Inputs=+-
  Rotated_Target_Id : Sum  Inputs=+-
  Rotated_Target_Iq : Sum  Inputs=|++
  TargetPhase_PU_Floor : Rounding
  TargetPhase_PU_Wrap : Sum  Inputs=+-
  TargetPhase_RadToPU : Gain  Gain=single(0.15915494)
  TargetPhase_SinCos_Service : YMBOX_SharedMath_Lib/SinCos_Service  SystemSampleTime=-1  VariantActivationTime=update diagram  AllowFlexibleInterface=on  Latency=0  AutoFrameSizeCalculation=off
  Target_Phase_Magnitude : Product  Inputs=**
  Target_Phase_Negate : Gain  Gain=single(-1)
  Unity : Constant  Value=single(1)
  targetId : Outport  OutDataTypeStr=single
  targetIq : Outport  Port=2  OutDataTypeStr=single
  wires:
  One_Minus_Blend/1 -> Target_Phase_Magnitude/1
  Unity/1 -> One_Minus_Blend/1
  Target_Phase_Magnitude/1 -> Target_Phase_Negate/1
  blendWeight/1 -> One_Minus_Blend/2
  elecAngleDeltaRad/1 -> Target_Phase_Magnitude/2
  Target_Phase_Negate/1 -> TargetPhase_RadToPU/1
  TargetPhase_RadToPU/1 -> TargetPhase_PU_Wrap/1, TargetPhase_PU_Floor/1
  TargetPhase_PU_Wrap/1 -> TargetPhase_SinCos_Service/1
  idRaw/1 -> Id_Cos/1, Id_Sin/1
  iqRaw/1 -> Iq_Sin/1, Iq_Cos/1
  TargetPhase_SinCos_Service/2 -> Iq_Sin/2, Id_Sin/2
  TargetPhase_SinCos_Service/1 -> Iq_Cos/2, Id_Cos/2
  Id_Sin/1 -> Rotated_Target_Iq/1
  Iq_Cos/1 -> Rotated_Target_Iq/2
  Id_Cos/1 -> Rotated_Target_Id/1
  Iq_Sin/1 -> Rotated_Target_Id/2
  Rotated_Target_Iq/1 -> targetIq/1
  Rotated_Target_Id/1 -> targetId/1
  TargetPhase_PU_Floor/1 -> TargetPhase_PU_Wrap/2

== system YMBOX_Control_Core/MDTM/MDTM/MDTM_SMO/SMO_Handover_SeedEstimator/Handover_Current_Frame_Transform ==
  blendWeight : Inport  OutDataTypeStr=single
  elecAngleDeltaRad : Inport  Port=2  OutDataTypeStr=single
  controlElecAngleRad : Inport  Port=3  OutDataTypeStr=single
  phaseU : Inport  Port=4  OutDataTypeStr=single
  phaseV : Inport  Port=5  OutDataTypeStr=single
  phaseW : Inport  Port=6  OutDataTypeStr=single
  Compute_Enable : EnablePort  OutDataTypeStr=boolean
  Clarke_Alpha_Gain : Gain  Gain=single(0.6666666)  ParamDataTypeStr=single  OutDataTypeStr=single
  Clarke_Alpha_Sum : Sum  Inputs=+--
  Clarke_Beta_Difference : Sum  Inputs=+-
  Clarke_Beta_Gain : Gain  Gain=single(0.5773502)  ParamDataTypeStr=single  OutDataTypeStr=single
  ControlAngle_PU_Floor : Rounding
  ControlAngle_PU_Wrap : Sum  Inputs=+-  OutDataTypeStr=single
  ControlAngle_RadToPU : Gain  Gain=single(0.15915494)  ParamDataTypeStr=single  OutDataTypeStr=single
  ControlAngle_SinCos_Service : YMBOX_SharedMath_Lib/SinCos_Service  SystemSampleTime=-1  VariantActivationTime=update diagram  AllowFlexibleInterface=on  Latency=0  AutoFrameSizeCalculation=off
  Control_Id : Sum  Inputs=|++
  Control_Id_Alpha : Product  Inputs=**
  Control_Id_Beta : Product  Inputs=**
  Control_Iq : Sum  Inputs=+-
  Control_Iq_Alpha : Product  Inputs=**
  Control_Iq_Beta : Product  Inputs=**
  Half_PhaseV : Gain  Gain=single(0.5)  ParamDataTypeStr=single  OutDataTypeStr=single
  Half_PhaseW : Gain  Gain=single(0.5)  ParamDataTypeStr=single  OutDataTypeStr=single
  ObserverAngle_PU_Floor : Rounding
  ObserverAngle_PU_Wrap : Sum  Inputs=+-  OutDataTypeStr=single
  ObserverAngle_RadToPU : Gain  Gain=single(0.15915494)  ParamDataTypeStr=single  OutDataTypeStr=single
  ObserverAngle_SinCos_Service : YMBOX_SharedMath_Lib/SinCos_Service  SystemSampleTime=-1  VariantActivationTime=update diagram  AllowFlexibleInterface=on  Latency=0  AutoFrameSizeCalculation=off
  Observer_Angle_Offset : Product  Inputs=**
  Observer_Frame_Angle : Sum  Inputs=+-
  Observer_Iq : Sum  Inputs=+-
  Observer_Iq_Alpha : Product  Inputs=**
  Observer_Iq_Beta : Product  Inputs=**
  One_Minus_Blend : Sum  Inputs=+-
  Unity : Constant  Value=single(1)  OutDataTypeStr=single
  iAlpha : Outport
  iBeta : Outport  Port=2
  idCtrl : Outport  Port=3
  iqCtrl : Outport  Port=4
  iqObs : Outport  Port=5
  wires:
  Observer_Iq_Alpha/1 -> Observer_Iq/2
  Unity/1 -> One_Minus_Blend/1
  One_Minus_Blend/1 -> Observer_Angle_Offset/1
  Observer_Angle_Offset/1 -> Observer_Frame_Angle/2
  ControlAngle_RadToPU/1 -> ControlAngle_PU_Wrap/1, ControlAngle_PU_Floor/1
  Observer_Frame_Angle/1 -> ObserverAngle_RadToPU/1
  Observer_Iq_Beta/1 -> Observer_Iq/1
  ObserverAngle_RadToPU/1 -> ObserverAngle_PU_Wrap/1, ObserverAngle_PU_Floor/1
  ControlAngle_PU_Wrap/1 -> ControlAngle_SinCos_Service/1
  Clarke_Beta_Difference/1 -> Clarke_Beta_Gain/1
  Half_PhaseV/1 -> Clarke_Alpha_Sum/2
  Half_PhaseW/1 -> Clarke_Alpha_Sum/3
  Clarke_Alpha_Sum/1 -> Clarke_Alpha_Gain/1
  ObserverAngle_PU_Wrap/1 -> ObserverAngle_SinCos_Service/1
  ControlAngle_SinCos_Service/2 -> Control_Id_Beta/2, Control_Iq_Alpha/2
  ControlAngle_SinCos_Service/1 -> Control_Iq_Beta/2, Control_Id_Alpha/2
  Clarke_Beta_Gain/1 -> iBeta/1, Control_Id_Beta/1, Control_Iq_Beta/1, Observer_Iq_Beta/1
  Clarke_Alpha_Gain/1 -> iAlpha/1, Observer_Iq_Alpha/1, Control_Id_Alpha/1, Control_Iq_Alpha/1
  ObserverAngle_SinCos_Service/2 -> Observer_Iq_Alpha/2
  ObserverAngle_SinCos_Service/1 -> Observer_Iq_Beta/2
  Control_Id_Alpha/1 -> Control_Id/1
  Control_Id_Beta/1 -> Control_Id/2
  Control_Iq_Beta/1 -> Control_Iq/1
  Control_Iq_Alpha/1 -> Control_Iq/2
  Control_Id/1 -> idCtrl/1
  Control_Iq/1 -> iqCtrl/1
  Observer_Iq/1 -> iqObs/1
  elecAngleDeltaRad/1 -> Observer_Angle_Offset/2
  controlElecAngleRad/1 -> Observer_Frame_Angle/1, ControlAngle_RadToPU/1
  phaseU/1 -> Clarke_Alpha_Sum/1
  phaseV/1 -> Half_PhaseV/1, Clarke_Beta_Difference/1
  phaseW/1 -> Half_PhaseW/1, Clarke_Beta_Difference/2
  blendWeight/1 -> One_Minus_Blend/2
  ControlAngle_PU_Floor/1 -> ControlAngle_PU_Wrap/2
  ObserverAngle_PU_Floor/1 -> ObserverAngle_PU_Wrap/2

== system YMBOX_Control_Core/MDSA/MDSA_Subsystem/PwmOutput/PwmEnable/SVM/SectorCalc ==
  VfMDSA_VoltAlpha_V : Inport
  VfMDSA_VoltBeta_V : Inport  Port=2
  Constant : Constant  Value=1/sqrt(3)  OutDataTypeStr=single
  If : If  IfExpression=u1 < 0
  If Action Subsystem : Subsystem  TreatAsAtomicUnit=on
  If Action Subsystem1 : Subsystem  TreatAsAtomicUnit=on
  Merge : Merge
  Product : Product
  VeMDSA_Sector_enum : Outport
  wires:
  Merge/1 -> VeMDSA_Sector_enum/1  "VeMDSA_Sector_enum"
  If Action Subsystem/1(Out1) -> Merge/2
  If Action Subsystem1/1(Out1) -> Merge/1
  If/1 -> If Action Subsystem/Action
  If/2 -> If Action Subsystem1/Action
  VfMDSA_VoltAlpha_V/1 -> If Action Subsystem1/2(In1), If Action Subsystem/1(In1)
  Product/1 -> If Action Subsystem1/1(In2), If Action Subsystem/2(In2)
  Constant/1 -> Product/2
  VfMDSA_VoltBeta_V/1 -> Product/1, If/1

== system YMBOX_Control_Core/MDSA/MDSA_Subsystem/PwmOutput/PwmEnable/SVM/T1T2CoefCalc ==
  VeMDSA_Sector_enum : Inport
  VfMDSA_VoltAlpha_V : Inport  Port=2
  VfMDSA_VoltBeta_V : Inport  Port=3
  VfMDSA_DCBusVolt_V : Inport  Port=4
  Add : Sum
  Constant : Constant  Value=KfMDSA_MaxDuty_NULL-KfMDSA_MinDuty_NULL  OutDataTypeStr=single
  Demux : Demux  Outputs=2
  If : If  NumInputs=2  IfExpression=u1 <= u2
  If Action Subsystem : Subsystem  TreatAsAtomicUnit=on
  If Action Subsystem1 : Subsystem  TreatAsAtomicUnit=on
  Merge : Merge  Inputs=6
  Merge1 : Merge
  Merge2 : Merge
  Merge3 : Merge
  Mux{,1..5} (6 alike) : Mux  Inputs=2
  Saturation : Saturate  UpperLimit=inf  LowerLimit=0
  Saturation1 : Saturate  UpperLimit=inf  LowerLimit=0
  Switch Case : SwitchCase  CaseConditions={1,2,3,4,5,6}  ShowDefaultCase=off
  Switch Case Action Subsystem : Subsystem  TreatAsAtomicUnit=on
  Switch Case Action Subsystem1 : Subsystem  TreatAsAtomicUnit=on
  Switch Case Action Subsystem2 : Subsystem  TreatAsAtomicUnit=on
  Switch Case Action Subsystem3 : Subsystem  TreatAsAtomicUnit=on
  Switch Case Action Subsystem4 : Subsystem  TreatAsAtomicUnit=on
  Switch Case Action Subsystem5 : Subsystem  TreatAsAtomicUnit=on
  VfMDSA_T1Coef_NULL : Outport
  VfMDSA_T2Coef_NULL : Outport  Port=2
  VfMDSA_k_svm_NULL : Outport  Port=3
  wires:
  If Action Subsystem1/3(Out3) -> Merge3/2
  If Action Subsystem/3(Out3) -> Merge3/1
  If Action Subsystem1/2(Out2) -> Merge2/2
  If Action Subsystem/2(Out2) -> Merge2/1
  If Action Subsystem1/1(Out1) -> Merge1/2
  If Action Subsystem/1(Out1) -> Merge1/1
  Saturation1/1 -> If Action Subsystem/2(In2), If Action Subsystem1/2(In2), Add/2
  Saturation/1 -> Add/1, If Action Subsystem/1(In1), If Action Subsystem1/1(In1)
  Merge3/1 -> VfMDSA_k_svm_NULL/1  "VfMDSA_k_svm_NULL"
  If/1 -> If Action Subsystem/Action
  If/2 -> If Action Subsystem1/Action
  Add/1 -> If/1
  Merge/1 -> Demux/1
  Demux/2 -> Saturation1/1
  Demux/1 -> Saturation/1
  Mux5/1 -> Merge/6
  Mux4/1 -> Merge/5
  Mux3/1 -> Merge/4
  Mux2/1 -> Merge/3
  Mux/1 -> Merge/2
  Mux1/1 -> Merge/1
  Switch Case Action Subsystem/2(VfMDSA_tmpT2Coef_NULL) -> Mux5/2
  Switch Case Action Subsystem/1(VfMDSA_tmpT1Coef_NULL) -> Mux5/1
  Switch Case Action Subsystem1/2(VfMDSA_tmpT2Coef_NULL) -> Mux4/2
  Switch Case Action Subsystem1/1(VfMDSA_tmpT1Coef_NULL) -> Mux4/1
  Switch Case Action Subsystem2/2(VfMDSA_tmpT2Coef_NULL) -> Mux3/2
  Switch Case Action Subsystem2/1(VfMDSA_tmpT1Coef_NULL) -> Mux3/1
  Switch Case Action Subsystem3/2(VfMDSA_tmpT2Coef_NULL) -> Mux2/2
  Switch Case Action Subsystem3/1(VfMDSA_tmpT1Coef_NULL) -> Mux2/1
  Switch Case Action Subsystem5/2(VfMDSA_tmpT2Coef_NULL) -> Mux1/2
  Switch Case Action Subsystem5/1(VfMDSA_tmpT1Coef_NULL) -> Mux1/1
  Switch Case Action Subsystem4/2(VfMDSA_tmpT2Coef_NULL) -> Mux/2
  Switch Case Action Subsystem4/1(VfMDSA_tmpT1Coef_NULL) -> Mux/1
  Switch Case/1 -> Switch Case Action Subsystem/Action
  Switch Case/2 -> Switch Case Action Subsystem1/Action
  Switch Case/3 -> Switch Case Action Subsystem2/Action
  Switch Case/4 -> Switch Case Action Subsystem3/Action
  Switch Case/5 -> Switch Case Action Subsystem4/Action
  Switch Case/6 -> Switch Case Action Subsystem5/Action
  VfMDSA_DCBusVolt_V/1 -> Switch Case Action Subsystem3/3(VfMDSA_DCBusVolt_V), Switch Case Action Subsystem2/3(VuMDSA_DCBusVolt_V), Switch Case Action Subsystem1/3(VfMDSA_DCBusVolt_V), Switch Case Action Subsystem/3(VfMDSA_DCBusVolt_V), Switch Case Action Subsystem4/3(VfMDSA_DCBusVolt_V), Switch Case Action Subsystem5/3(VfMDSA_DCBusVolt_V)
  VfMDSA_VoltBeta_V/1 -> Switch Case Action Subsystem3/2(VfMDSA_VoltBeta_V), Switch Case Action Subsystem2/2(VfMDSA_VoltBeta_V), Switch Case Action Subsystem1/2(VfMDSA_VoltBeta_V), Switch Case Action Subsystem/2(VfMDSA_VoltBeta_V), Switch Case Action Subsystem4/2(VfMDSA_VoltBeta_V), Switch Case Action Subsystem5/2(VfMDSA_VoltBeta_V)
  VfMDSA_VoltAlpha_V/1 -> Switch Case Action Subsystem4/1(VfMDSA_VoltAlpha_V), Switch Case Action Subsystem3/1(VfMDSA_VoltAlpha_V), Switch Case Action Subsystem2/1(VfMDSA_VoltAlpha_V), Switch Case Action Subsystem1/1(VfMDSA_VoltAlpha_V), Switch Case Action Subsystem/1(VfMDSA_VoltAlpha_V), Switch Case Action Subsystem5/1(VfMDSA_VoltAlpha_V)
  VeMDSA_Sector_enum/1 -> Switch Case/1
  Merge1/1 -> VfMDSA_T1Coef_NULL/1  "VfMDSA_T1Coef_NULL"
  Merge2/1 -> VfMDSA_T2Coef_NULL/1  "VfMDSA_T2Coef_NULL"
  Constant/1 -> If/2

== system YMBOX_Control_Core/MDSA/MDSA_Subsystem/PwmOutput/PwmEnable/SVM/TonUVWCal ==
  VeMDSA_Sector_enum : Inport
  VfMDSA_T1Coef_NULL : Inport  Port=2
  VfMDSA_T2Coef_NULL : Inport  Port=3
  Add : Sum  Inputs=+++
  Add1 : Sum  Inputs=+-+
  Add2 : Sum  Inputs=+--
  Constant : Constant  Value=KfMDSA_MaxDuty_NULL+KfMDSA_MinDuty_NULL  OutDataTypeStr=single
  Demux1 : Demux  Outputs=3
  Gain : Gain  Gain=0.5  OutDataTypeStr=single
  Gain1 : Gain  Gain=0.5  OutDataTypeStr=single
  Gain2 : Gain  Gain=0.5  OutDataTypeStr=single
  Merge : Merge  Inputs=6
  Mux{1..6} (6 alike) : Mux  Inputs=3
  Saturation : Saturate  UpperLimit=KfMDSA_MaxDuty_NULL  LowerLimit=KfMDSA_MinDuty_NULL  OutMin=0  OutMax=1
  Saturation1 : Saturate  UpperLimit=KfMDSA_MaxDuty_NULL  LowerLimit=KfMDSA_MinDuty_NULL  OutMin=0  OutMax=1
  Saturation2 : Saturate  UpperLimit=KfMDSA_MaxDuty_NULL  LowerLimit=KfMDSA_MinDuty_NULL  OutMin=0  OutMax=1
  Signal Conversion : SignalConversion  OverrideOpt=off
  Signal Conversion1 : SignalConversion  OverrideOpt=off
  Signal Conversion2 : SignalConversion  OverrideOpt=off
  Switch Case : SwitchCase  CaseConditions={1,2,3,4,5,6}  ShowDefaultCase=off
  Switch Case Action Subsystem : Subsystem  TreatAsAtomicUnit=on
  Switch Case Action Subsystem1 : Subsystem  TreatAsAtomicUnit=on
  Switch Case Action Subsystem2 : Subsystem  TreatAsAtomicUnit=on
  Switch Case Action Subsystem3 : Subsystem  TreatAsAtomicUnit=on
  Switch Case Action Subsystem4 : Subsystem  TreatAsAtomicUnit=on
  Switch Case Action Subsystem5 : Subsystem  TreatAsAtomicUnit=on
  VfMDSA_PwmDutyCyclePhaseU_NULL : Outport
  VfMDSA_PwmDutyCyclePhaseV_NULL : Outport  Port=2
  VfMDSA_PwmDutyCyclePhaseW_NULL : Outport  Port=3
  wires:
  Saturation2/1 -> Signal Conversion2/1
  Demux1/3 -> Saturation2/1
  Saturation1/1 -> Signal Conversion1/1
  Demux1/2 -> Saturation1/1
  Saturation/1 -> Signal Conversion/1
  Demux1/1 -> Saturation/1
  Signal Conversion2/1 -> VfMDSA_PwmDutyCyclePhaseW_NULL/1
  Signal Conversion1/1 -> VfMDSA_PwmDutyCyclePhaseV_NULL/1
  Signal Conversion/1 -> VfMDSA_PwmDutyCyclePhaseU_NULL/1
  Merge/1 -> Demux1/1
  Mux6/1 -> Merge/6
  Mux5/1 -> Merge/5
  Mux4/1 -> Merge/4
  Mux3/1 -> Merge/3
  Mux2/1 -> Merge/2
  Mux1/1 -> Merge/1
  Switch Case Action Subsystem/3(VfMDSA_PwmDutyCyclePhaseW_NULL) -> Mux6/3
  Switch Case Action Subsystem/2(VfMDSA_PwmDutyCyclePhaseV_NULL) -> Mux6/2
  Switch Case Action Subsystem/1(VfMDSA_PwmDutyCyclePhaseU_NULL) -> Mux6/1
  Switch Case Action Subsystem1/3(VfMDSA_PwmDutyCyclePhaseW_NULL) -> Mux5/3
  Switch Case Action Subsystem1/2(VfMDSA_PwmDutyCyclePhaseV_NULL) -> Mux5/2
  Switch Case Action Subsystem1/1(VfMDSA_PwmDutyCyclePhaseU_NULL) -> Mux5/1
  Switch Case Action Subsystem2/3(VfMDSA_PwmDutyCyclePhaseW_NULL) -> Mux4/3
  Switch Case Action Subsystem2/2(VfMDSA_PwmDutyCyclePhaseV_NULL) -> Mux4/2
  Switch Case Action Subsystem2/1(VfMDSA_PwmDutyCyclePhaseU_NULL) -> Mux4/1
  Switch Case Action Subsystem3/3(VfMDSA_PwmDutyCyclePhaseW_NULL) -> Mux3/3
  Switch Case Action Subsystem3/2(VfMDSA_PwmDutyCyclePhaseV_NULL) -> Mux3/2
  Switch Case Action Subsystem3/1(VfMDSA_PwmDutyCyclePhaseU_NULL) -> Mux3/1
  Switch Case Action Subsystem4/3(VfMDSA_PwmDutyCyclePhaseW_NULL) -> Mux2/3
  Switch Case Action Subsystem4/2(VfMDSA_PwmDutyCyclePhaseV_NULL) -> Mux2/2
  Switch Case Action Subsystem4/1(VfMDSA_PwmDutyCyclePhaseU_NULL) -> Mux2/1
  Switch Case Action Subsystem5/3(VfMDSA_PwmDutyCyclePhaseW_NULL) -> Mux1/3
  Switch Case Action Subsystem5/2(VfMDSA_PwmDutyCyclePhaseV_NULL) -> Mux1/2
  Switch Case Action Subsystem5/1(VfMDSA_PwmDutyCyclePhaseU_NULL) -> Mux1/1
  Switch Case/1 -> Switch Case Action Subsystem/Action
  Switch Case/2 -> Switch Case Action Subsystem1/Action
  Switch Case/3 -> Switch Case Action Subsystem2/Action
  Switch Case/4 -> Switch Case Action Subsystem3/Action
  Switch Case/5 -> Switch Case Action Subsystem4/Action
  Switch Case/6 -> Switch Case Action Subsystem5/Action
  Gain2/1 -> Switch Case Action Subsystem5/3(VfMDSA_PwmDutyCyclePhaseC_NULL), Switch Case Action Subsystem4/3(VfMDSA_PwmDutyCyclePhaseC_NULL), Switch Case Action Subsystem3/3(VfMDSA_PwmDutyCyclePhaseC_NULL), Switch Case Action Subsystem2/3(VfMDSA_PwmDutyCyclePhaseC_NULL), Switch Case Action Subsystem/3(VfMDSA_PwmDutyCyclePhaseC_NULL), Switch Case Action Subsystem1/3(VfMDSA_PwmDutyCyclePhaseC_NULL1)
  Gain1/1 -> Switch Case Action Subsystem4/2(VfMDSA_PwmDutyCyclePhaseB_NULL), Switch Case Action Subsystem2/2(VfMDSA_PwmDutyCyclePhaseB_NULL), Switch Case Action Subsystem/2(VfMDSA_PwmDutyCyclePhaseB_NULL), Switch Case Action Subsystem1/2(VfMDSA_PwmDutyCyclePhaseB_NULL), Switch Case Action Subsystem3/2(VfMDSA_PwmDutyCyclePhaseB_NULL), Switch Case Action Subsystem5/2(VfMDSA_PwmDutyCyclePhaseB_NULL)
  Gain/1 -> Switch Case Action Subsystem4/1(VfMDSA_PwmDutyCyclePhaseA_NULL), Switch Case Action Subsystem3/1(VfMDSA_PwmDutyCyclePhaseA_NULL), Switch Case Action Subsystem1/1(VfMDSA_PwmDutyCyclePhaseA_NULL), Switch Case Action Subsystem/1(VfMDSA_PwmDutyCyclePhaseA_NULL), Switch Case Action Subsystem2/1(VfMDSA_PwmDutyCyclePhaseA_NULL), Switch Case Action Subsystem5/1(VfMDSA_PwmDutyCyclePhaseA_NULL)
  VeMDSA_Sector_enum/1 -> Switch Case/1
  Add2/1 -> Gain2/1
  Add1/1 -> Gain1/1
  Add/1 -> Gain/1
  VfMDSA_T2Coef_NULL/1 -> Add/3, Add1/3, Add2/3
  VfMDSA_T1Coef_NULL/1 -> Add/2, Add1/2, Add2/2
  Constant/1 -> Add/1, Add1/1, Add2/1

== system YMBOX_Control_Core/MDSA/MDSA_Subsystem/UalphaUbetaCalc/Subsystem/UalphaUbetaCalc1/ElecAngle_Advance_SinCos ==
  VfMDSA_MotElecAngle_rad : Inport
  VfMDSA_MotElecSpd_rads : Inport  Port=2
  VfMDSA_PwmFreq_Hz : Inport  Port=3
  Add_ElecAngle_Advance_Rad : Sum  OutDataTypeStr=single  AccumDataTypeStr=single  RndMeth=Nearest  SaturateOnIntegerOverflow=on
  Constant1 : Constant  Value=KfMDSA_EAngleCompScale_NULL  OutDataTypeStr=single
  ElecAngle_Rad_To_Pu : Product  Inputs=*/
  ElecAngle_To_Single : DataTypeConversion  OutDataTypeStr=single
  ElecSpeed_PerPwmTick_Rad : Product  Inputs=*/
  Scale_ElecAngle_Advance_Rad : Product
  SinCos_Service : YMBOX_SharedMath_Lib/SinCos_Service  SystemSampleTime=-1  VariantActivationTime=update diagram  AllowFlexibleInterface=on  Latency=0  AutoFrameSizeCalculation=off
  Two_Pi_Rad_Mod : Constant  Value=single(2*pi)  OutDataTypeStr=single
  Two_Pi_Rad_Normalize : Constant  Value=single(2*pi)  OutDataTypeStr=single
  Wrap_ElecAngle_Rad : Math  Operator=mod  SignedPower=on  OutMin=0  OutMax=2*pi  RndMeth=Nearest
  VfMDSA_EAngleEstimatedCos_NULL : Outport
  VfMDSA_EAngleEstimatedSin_NULL : Outport  Port=2
  wires:
  Constant1/1 -> Scale_ElecAngle_Advance_Rad/2
  VfMDSA_MotElecAngle_rad/1 -> Add_ElecAngle_Advance_Rad/1
  VfMDSA_PwmFreq_Hz/1 -> ElecSpeed_PerPwmTick_Rad/2
  ElecAngle_To_Single/1 -> ElecAngle_Rad_To_Pu/1
  Two_Pi_Rad_Normalize/1 -> ElecAngle_Rad_To_Pu/2
  ElecAngle_Rad_To_Pu/1 -> SinCos_Service/1
  SinCos_Service/1 -> VfMDSA_EAngleEstimatedCos_NULL/1
  SinCos_Service/2 -> VfMDSA_EAngleEstimatedSin_NULL/1
  ElecSpeed_PerPwmTick_Rad/1 -> Scale_ElecAngle_Advance_Rad/1
  Scale_ElecAngle_Advance_Rad/1 -> Add_ElecAngle_Advance_Rad/2
  VfMDSA_MotElecSpd_rads/1 -> ElecSpeed_PerPwmTick_Rad/1
  Add_ElecAngle_Advance_Rad/1 -> Wrap_ElecAngle_Rad/1
  Two_Pi_Rad_Mod/1 -> Wrap_ElecAngle_Rad/2
  Wrap_ElecAngle_Rad/1 -> ElecAngle_To_Single/1

== system YMBOX_Control_Core/MDSA/MDSA_Subsystem/UalphaUbetaCalc/Subsystem/UalphaUbetaCalc1/IPark ==
  VfMDSA_VoltD_V : Inport
  VfMDSA_VoltQ_V : Inport  Port=2
  VfMDSA_EAngleEstimatedCos_NULL : Inport  Port=3
  VfMDSA_EAngleEstimatedSin_NULL : Inport  Port=4
  Product{,1..3} (4 alike) : Product
  Subtract : Sum  Inputs=+-
  Subtract1 : Sum
  VfMDSA_VoltAlpha_V : Outport
  VfMDSA_VoltBeta_V : Outport  Port=2
  wires:
  Subtract1/1 -> VfMDSA_VoltBeta_V/1
  Product3/1 -> Subtract1/2
  Product2/1 -> Subtract1/1
  Subtract/1 -> VfMDSA_VoltAlpha_V/1
  Product1/1 -> Subtract/2
  Product/1 -> Subtract/1
  VfMDSA_EAngleEstimatedSin_NULL/1 -> Product2/2, Product1/2
  VfMDSA_VoltQ_V/1 -> Product3/1, Product1/1
  VfMDSA_EAngleEstimatedCos_NULL/1 -> Product3/2, Product/2
  VfMDSA_VoltD_V/1 -> Product/1, Product2/1

== system YMBOX_Control_Core/MDSA/MDSA_Subsystem/PwmOutput/PwmEnable/SVM/SectorCalc/If Action Subsystem ==
  In1 : Inport
  In2 : Inport  Port=2
  Action Port : ActionPort  ActionPortLabel=if(u1 < 0)
  Constant : Constant  Value=4  OutDataTypeStr=uint8
  Constant1 : Constant  Value=6  OutDataTypeStr=uint8
  Constant2 : Constant  Value=5  OutDataTypeStr=uint8
  Relational Operator : RelationalOperator  Operator=<=  OutDataTypeStr=boolean  InputSameDT=off
  Relational Operator1 : RelationalOperator  Operator=>  OutDataTypeStr=boolean  InputSameDT=off
  Switch : Switch  Criteria=u2 ~= 0  SaturateOnIntegerOverflow=off  InputSameDT=off
  Switch1 : Switch  Criteria=u2 ~= 0  SaturateOnIntegerOverflow=off  InputSameDT=off
  Unary Minus : UnaryMinus
  Out1 : Outport
  wires:
  Relational Operator1/1 -> Switch1/2
  Constant2/1 -> Switch1/3
  In2/1 -> Relational Operator/2, Unary Minus/1
  Switch/1 -> Out1/1
  Switch1/1 -> Switch/3
  Constant1/1 -> Switch1/1
  Unary Minus/1 -> Relational Operator1/2
  Relational Operator/1 -> Switch/2
  Constant/1 -> Switch/1
  In1/1 -> Relational Operator/1, Relational Operator1/1
